simulink model "bb_simscape"  (R2025b)
settings: Solver=ode23t  StartTime=0.0  StopTime=19  MaxStep=2e-3  RelTol=1e-4
model workspace (MAT data in the model file):
  P_C = 343
  P_LAT_US = 200
  P_MAX_MM = 1000
  P_MIN_MM = 20
  P_MM_PER_US_Q16 = 11239
  P_NOISE_MM = 2
  P_R = 0.02
  P_SEED = 12345
  P_TS = 0.0001
values from neighbouring files (symbols this model uses):
  m = bb_metrics(o, scn)    [run_verification.m]    (also in sweep_ki.m)
  s = Simulink.HMI.ParamSourceInfo    [build_bb_live.m]    (also in build_bb_simscape.m = pl; export_motion_csv.m = interp1(o.s_m.Time, squeeze(o.s_m.Data), t, 'linear', 'extra; hcsr04_model.m = uint32(mod(1664525*double(s) + 1013904223, 4294967296)); test_rolling.m = mdl)
undefined symbols (not defined in the file or in its folder): X, Y, Z
libraries: sm_lib x41, nesl_utility x7
(part 2 of 2)

== matlab function bb_simscape/FPGA_Controller/pid_ctrl ==
  settings: fimath=hdlfimath
  data: pos_mm input uint16; servo_us output uint16; sample input boolean; setpoint input uint16; kp input uint16; ki input uint16; kd input uint16; center input uint16; smin input uint16; smax input uint16; mode input uint16; manual_us input uint16; dshift input uint16; ilim input uint16; int_rst input boolean; err_mm output int16; iterm output int16; dterm output int16; ctl_done output boolean
function [servo_us, err_mm, iterm, dterm, ctl_done] = pid_ctrl(pos_mm, sample, setpoint, kp, ki, kd, ...
    center, smin, smax, mode, manual_us, dshift, ilim, int_rst)
%PID_CTRL  Discrete PID, executed once per sensor sample (4-cycle sequence,
%   one shared multiplier).
%     e  = setpoint - pos                     [mm]
%     P  = Kp*e
%     I += Ki*e,  clamped to +/- ilim us      (anti-windup)
%     D  = Kd*filt(pos[k-1]-pos[k])           (derivative on measurement,
%                                              IIR alpha = 1/2^dshift)
%     servo = clamp(center +/- (P+I+D), smin, smax)
%   Gains are Q8.8; internal sums are in us*256.
%   mode bit0 = loop enable (else servo = manual_us), bit1 = invert output.
%   Bit-exact sample-level reference: bb_ctrl_ref.m.
%#codegen
persistent stg have pos_prev df e_r iacc pacc dacc servo_r err_r it_r dt_r done_r
if isempty(stg)
    stg = uint8(0); have = false; pos_prev = uint16(0); df = int32(0); e_r = int32(0);
    iacc = int32(0); pacc = int32(0); dacc = int32(0);
    servo_r = uint16(1750); err_r = int16(0); it_r = int16(0); dt_r = int16(0); done_r = false;
end
servo_us = servo_r;
err_mm   = err_r;
iterm    = it_r;
dterm    = dt_r;
ctl_done = done_r;

done_r = false;
enable = bitand(mode, uint16(1)) ~= uint16(0);
invert = bitand(mode, uint16(2)) ~= uint16(0);

% ---- shared multiplier: operand select by stage ----
if stg == uint8(1)
    ma = int32(kp);  mb = e_r;
elseif stg == uint8(2)
    ma = int32(ki);  mb = e_r;
else
    ma = int32(kd);  mb = df;
end
prod = ma * mb;

if stg == uint8(0)
    if sample
        e = int32(setpoint) - int32(pos_mm);
        if e > int32(2000), e = int32(2000); end
        if e < int32(-2000), e = int32(-2000); end
        if have
            dm = int32(pos_prev) - int32(pos_mm);
        else
            dm = int32(0);
        end
        if dm > int32(127), dm = int32(127); end
        if dm < int32(-127), dm = int32(-127); end
        have = true;
        pos_prev = pos_mm;
        x = dm*int32(256) - df;
        if dshift == uint16(0)
            df = df + x;
        elseif dshift == uint16(1)
            df = df + bitsra(x, 1);
        elseif dshift == uint16(2)
            df = df + bitsra(x, 2);
        elseif dshift == uint16(3)
            df = df + bitsra(x, 3);
        elseif dshift == uint16(4)
            df = df + bitsra(x, 4);
        elseif dshift == uint16(5)
            df = df + bitsra(x, 5);
        elseif dshift == uint16(6)
            df = df + bitsra(x, 6);
        else
            df = df + bitsra(x, 7);
        end
        e_r = e;
        stg = uint8(1);
    end
elseif stg == uint8(1)                  % P = Kp*e
    pacc = prod;
    stg = uint8(2);
elseif stg == uint8(2)                  % I += Ki*e
    lim = int32(ilim) * int32(256);
    inew = iacc + prod;
    if inew > lim, inew = lim; end
    if inew < -lim, inew = -lim; end
    if enable
        iacc = inew;
    else
        iacc = int32(0);
    end
    stg = uint8(3);
else                                    % 3: D = Kd*df, combine, clamp
    dacc = bitsra(prod, 8);
    u = bitsra(pacc + iacc + dacc, 8);
    if u > int32(4000), u = int32(4000); end
    if u < int32(-4000), u = int32(-4000); end
    if invert, u = -u; end
    if enable
        out = int32(center) + u;
    else
        out = int32(manual_us);
    end
    if out > int32(smax), out = int32(smax); end
    if out < int32(smin), out = int32(smin); end
    servo_r = uint16(out);
    err_r = int16(e_r);
    it_r  = int16(bitsra(iacc, 8));
    dv = bitsra(dacc, 8);
    if dv > int32(32767), dv = int32(32767); end
    if dv < int32(-32768), dv = int32(-32768); end
    dt_r = int16(dv);
    done_r = true;
    stg = uint8(0);
end
if int_rst
    iacc = int32(0);
end
end
